simulink model "RonTrap_fig11"  (R2022b)
settings: Solver=ode15s  StartTime=-14  StopTime=39  MaxStep=0.025  RelTol=1e-7  AbsTol=1e-8
settings Model: Creator=Greatlovers  LastModifiedBy=Greatlovers

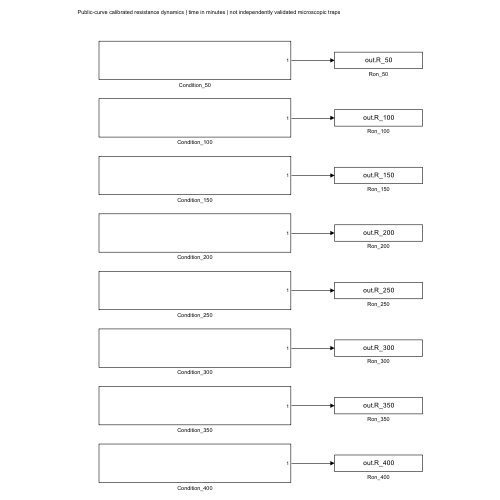
[thumbnail: Simulink's stored preview of the top-level diagram]
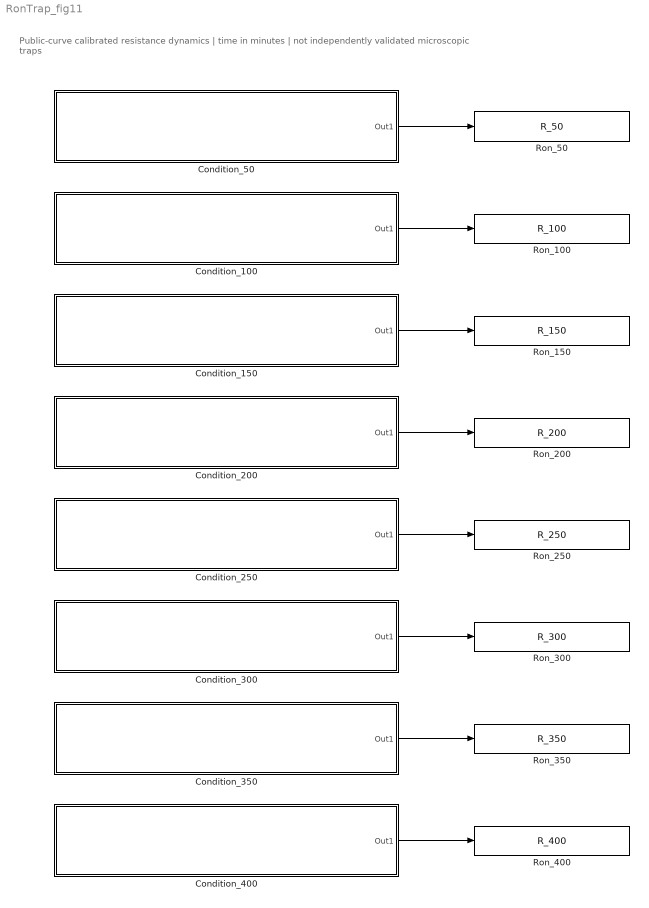
== system RonTrap_fig11 ==
  note: Public-curve calibrated resistance dynamics | time in minutes | not independently validated microscopic traps
  Condition_100 : Subsystem
  Condition_150 : Subsystem
  Condition_200 : Subsystem
  Condition_250 : Subsystem
  Condition_300 : Subsystem
  Condition_350 : Subsystem
  Condition_400 : Subsystem
  Condition_50 : Subsystem
  Ron_100 : ToWorkspace  VariableName=R_100  SaveFormat=Timeseries  SampleTime=-1
  Ron_150 : ToWorkspace  VariableName=R_150  SaveFormat=Timeseries  SampleTime=-1
  Ron_200 : ToWorkspace  VariableName=R_200  SaveFormat=Timeseries  SampleTime=-1
  Ron_250 : ToWorkspace  VariableName=R_250  SaveFormat=Timeseries  SampleTime=-1
  Ron_300 : ToWorkspace  VariableName=R_300  SaveFormat=Timeseries  SampleTime=-1
  Ron_350 : ToWorkspace  VariableName=R_350  SaveFormat=Timeseries  SampleTime=-1
  Ron_400 : ToWorkspace  VariableName=R_400  SaveFormat=Timeseries  SampleTime=-1
  Ron_50 : ToWorkspace  VariableName=R_50  SaveFormat=Timeseries  SampleTime=-1
  wires:
  Condition_50/1(Out1) -> Ron_50/1
  Condition_100/1(Out1) -> Ron_100/1
  Condition_150/1(Out1) -> Ron_150/1
  Condition_200/1(Out1) -> Ron_200/1
  Condition_250/1(Out1) -> Ron_250/1
  Condition_300/1(Out1) -> Ron_300/1
  Condition_350/1(Out1) -> Ron_350/1
  Condition_400/1(Out1) -> Ron_400/1

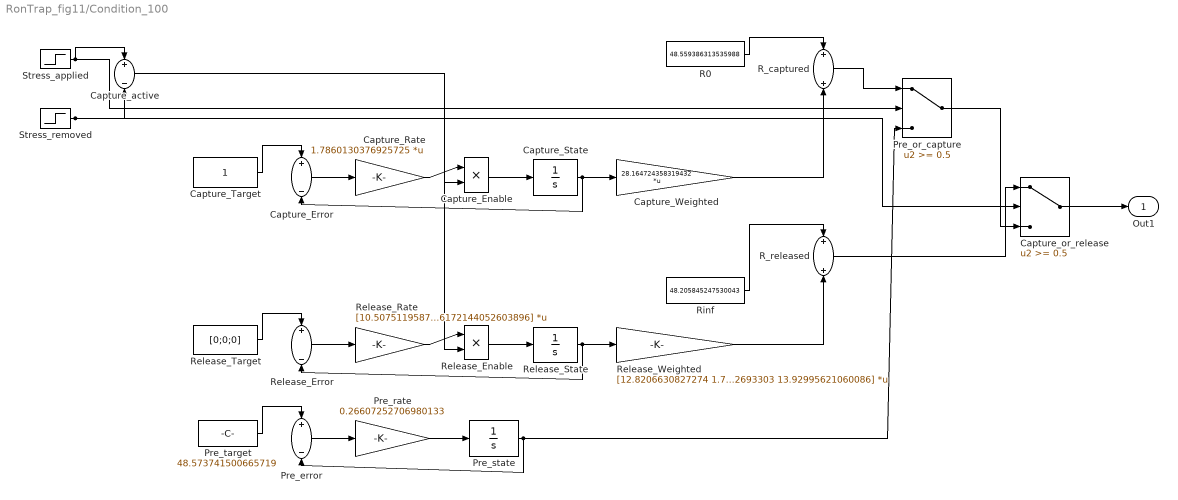
== system RonTrap_fig11/Condition_100 ==
  Capture_Enable : Product  Inputs=**
  Capture_Error : Sum  Inputs=+-
  Capture_Rate : Gain  Gain=1.7860130376925725  Multiplication=Matrix(K*u)
  Capture_State : Integrator
  Capture_Target : Constant
  Capture_Weighted : Gain  Gain=28.164724358319432  Multiplication=Matrix(K*u)
  Capture_active : Sum  Inputs=+-
  Capture_or_release : Switch  Threshold=0.5  SaturateOnIntegerOverflow=off  InputSameDT=off
  Pre_error : Sum  Inputs=+-
  Pre_or_capture : Switch  Threshold=0.5  SaturateOnIntegerOverflow=off  InputSameDT=off
  Pre_rate : Gain  Gain=0.26607252706980133
  Pre_state : Integrator  InitialCondition=47.988871358880552
  Pre_target : Constant  Value=48.573741500665719
  R0 : Constant  Value=48.559386313535988
  R_captured : Sum
  R_released : Sum
  Release_Enable : Product  Inputs=**
  Release_Error : Sum  Inputs=+-
  Release_Rate : Gain  Gain=[10.507511958742391 0 0;0 1.8533079959155121 0;0 0 0.26172144052603896]  Multiplication=Matrix(K*u)
  Release_State : Integrator  InitialCondition=[1;1;1]
  Release_Target : Constant  Value=[0;0;0]
  Release_Weighted : Gain  Gain=[12.8206630827274 1.7676461302693303 13.92995621060086]  Multiplication=Matrix(K*u)
  Rinf : Constant  Value=48.205845247530043
  Stress_applied : Step  Time=-0.066661845105779466  SampleTime=0
  Stress_removed : Step  Time=13.58333875417734  SampleTime=0
  Out1 : Outport
  wires:
  Stress_applied/1 -> Capture_active/1, Pre_or_capture/2
  Stress_removed/1 -> Capture_active/2, Release_Enable/2, Capture_or_release/2
  Capture_Target/1 -> Capture_Error/1
  Capture_State/1 -> Capture_Error/2, Capture_Weighted/1
  Capture_Error/1 -> Capture_Rate/1
  Capture_Rate/1 -> Capture_Enable/1
  Capture_Enable/1 -> Capture_State/1
  Release_Target/1 -> Release_Error/1
  Release_State/1 -> Release_Error/2, Release_Weighted/1
  Release_Error/1 -> Release_Rate/1
  Release_Rate/1 -> Release_Enable/1
  Release_Enable/1 -> Release_State/1
  Capture_active/1 -> Capture_Enable/2
  R0/1 -> R_captured/1
  Capture_Weighted/1 -> R_captured/2
  Rinf/1 -> R_released/1
  Release_Weighted/1 -> R_released/2
  Pre_target/1 -> Pre_error/1
  Pre_state/1 -> Pre_error/2, Pre_or_capture/3
  Pre_error/1 -> Pre_rate/1
  Pre_rate/1 -> Pre_state/1
  R_captured/1 -> Pre_or_capture/1
  R_released/1 -> Capture_or_release/1
  Pre_or_capture/1 -> Capture_or_release/3
  Capture_or_release/1 -> Out1/1

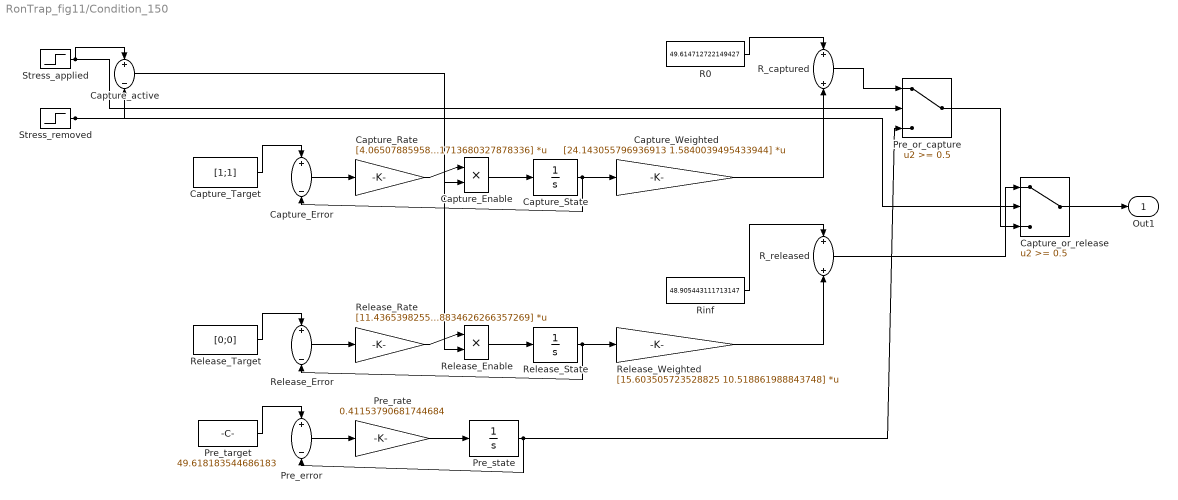
== system RonTrap_fig11/Condition_150 ==
  Capture_Enable : Product  Inputs=**
  Capture_Error : Sum  Inputs=+-
  Capture_Rate : Gain  Gain=[4.0650788595808649 0;0 0.11713680327878336]  Multiplication=Matrix(K*u)
  Capture_State : Integrator  InitialCondition=[0;0]
  Capture_Target : Constant  Value=[1;1]
  Capture_Weighted : Gain  Gain=[24.143055796936913 1.5840039495433944]  Multiplication=Matrix(K*u)
  Capture_active : Sum  Inputs=+-
  Capture_or_release : Switch  Threshold=0.5  SaturateOnIntegerOverflow=off  InputSameDT=off
  Pre_error : Sum  Inputs=+-
  Pre_or_capture : Switch  Threshold=0.5  SaturateOnIntegerOverflow=off  InputSameDT=off
  Pre_rate : Gain  Gain=0.41153790681744684
  Pre_state : Integrator  InitialCondition=48.544888767437868
  Pre_target : Constant  Value=49.618183544686183
  R0 : Constant  Value=49.614712722149427
  R_captured : Sum
  R_released : Sum
  Release_Enable : Product  Inputs=**
  Release_Error : Sum  Inputs=+-
  Release_Rate : Gain  Gain=[11.436539825510469 0;0 0.38834626266357269]  Multiplication=Matrix(K*u)
  Release_State : Integrator  InitialCondition=[1;1]
  Release_Target : Constant  Value=[0;0]
  Release_Weighted : Gain  Gain=[15.603505723528825 10.518861988843748]  Multiplication=Matrix(K*u)
  Rinf : Constant  Value=48.905443111713147
  Stress_applied : Step  Time=-0.066661845105779466  SampleTime=0
  Stress_removed : Step  Time=13.75000544608282  SampleTime=0
  Out1 : Outport
  wires:
  Stress_applied/1 -> Capture_active/1, Pre_or_capture/2
  Stress_removed/1 -> Capture_active/2, Release_Enable/2, Capture_or_release/2
  Capture_Target/1 -> Capture_Error/1
  Capture_State/1 -> Capture_Error/2, Capture_Weighted/1
  Capture_Error/1 -> Capture_Rate/1
  Capture_Rate/1 -> Capture_Enable/1
  Capture_Enable/1 -> Capture_State/1
  Release_Target/1 -> Release_Error/1
  Release_State/1 -> Release_Error/2, Release_Weighted/1
  Release_Error/1 -> Release_Rate/1
  Release_Rate/1 -> Release_Enable/1
  Release_Enable/1 -> Release_State/1
  Capture_active/1 -> Capture_Enable/2
  R0/1 -> R_captured/1
  Capture_Weighted/1 -> R_captured/2
  Rinf/1 -> R_released/1
  Release_Weighted/1 -> R_released/2
  Pre_target/1 -> Pre_error/1
  Pre_state/1 -> Pre_error/2, Pre_or_capture/3
  Pre_error/1 -> Pre_rate/1
  Pre_rate/1 -> Pre_state/1
  R_captured/1 -> Pre_or_capture/1
  R_released/1 -> Capture_or_release/1
  Pre_or_capture/1 -> Capture_or_release/3
  Capture_or_release/1 -> Out1/1

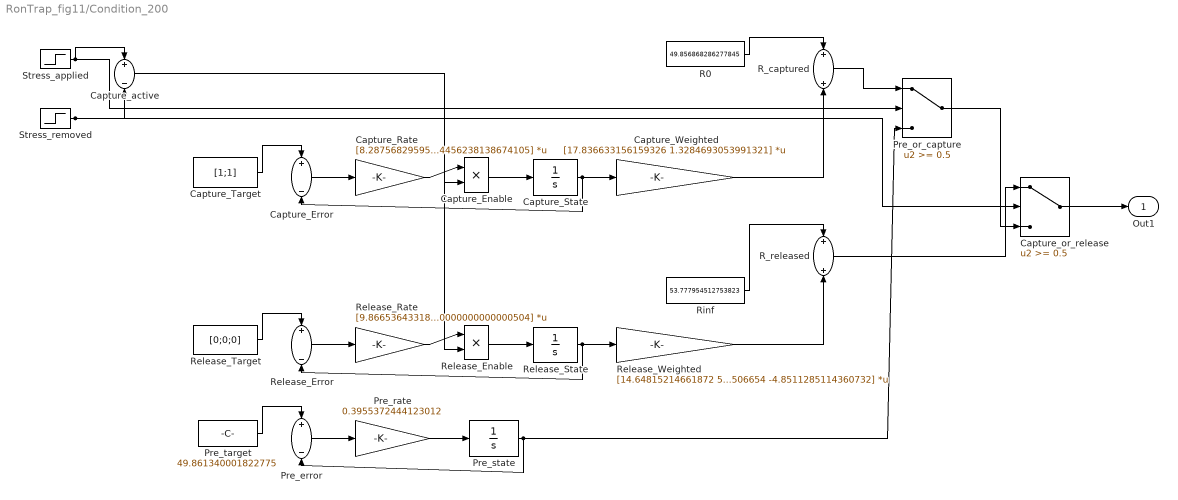
== system RonTrap_fig11/Condition_200 ==
  Capture_Enable : Product  Inputs=**
  Capture_Error : Sum  Inputs=+-
  Capture_Rate : Gain  Gain=[8.2875682959517381 0;0 0.24456238138674105]  Multiplication=Matrix(K*u)
  Capture_State : Integrator  InitialCondition=[0;0]
  Capture_Target : Constant  Value=[1;1]
  Capture_Weighted : Gain  Gain=[17.836633156159326 1.3284693053991321]  Multiplication=Matrix(K*u)
  Capture_active : Sum  Inputs=+-
  Capture_or_release : Switch  Threshold=0.5  SaturateOnIntegerOverflow=off  InputSameDT=off
  Pre_error : Sum  Inputs=+-
  Pre_or_capture : Switch  Threshold=0.5  SaturateOnIntegerOverflow=off  InputSameDT=off
  Pre_rate : Gain  Gain=0.3955372444123012
  Pre_state : Integrator  InitialCondition=48.754874141724315
  Pre_target : Constant  Value=49.861340001822775
  R0 : Constant  Value=49.856868286277845
  R_captured : Sum
  R_released : Sum
  Release_Enable : Product  Inputs=**
  Release_Error : Sum  Inputs=+-
  Release_Rate : Gain  Gain=[9.8665364331893439 0 0;0 0.56043585020711861 0;0 0 0.0050000000000000504]  Multiplication=Matrix(K*u)
  Release_State : Integrator  InitialCondition=[1;1;1]
  Release_Target : Constant  Value=[0;0;0]
  Release_Weighted : Gain  Gain=[14.64815214661872 5.4009738116506654 -4.8511285114360732]  Multiplication=Matrix(K*u)
  Rinf : Constant  Value=53.777954512753823
  Stress_applied : Step  Time=-0.066661845105779466  SampleTime=0
  Stress_removed : Step  Time=13.683338820821518  SampleTime=0
  Out1 : Outport
  wires:
  Stress_applied/1 -> Capture_active/1, Pre_or_capture/2
  Stress_removed/1 -> Capture_active/2, Release_Enable/2, Capture_or_release/2
  Capture_Target/1 -> Capture_Error/1
  Capture_State/1 -> Capture_Error/2, Capture_Weighted/1
  Capture_Error/1 -> Capture_Rate/1
  Capture_Rate/1 -> Capture_Enable/1
  Capture_Enable/1 -> Capture_State/1
  Release_Target/1 -> Release_Error/1
  Release_State/1 -> Release_Error/2, Release_Weighted/1
  Release_Error/1 -> Release_Rate/1
  Release_Rate/1 -> Release_Enable/1
  Release_Enable/1 -> Release_State/1
  Capture_active/1 -> Capture_Enable/2
  R0/1 -> R_captured/1
  Capture_Weighted/1 -> R_captured/2
  Rinf/1 -> R_released/1
  Release_Weighted/1 -> R_released/2
  Pre_target/1 -> Pre_error/1
  Pre_state/1 -> Pre_error/2, Pre_or_capture/3
  Pre_error/1 -> Pre_rate/1
  Pre_rate/1 -> Pre_state/1
  R_captured/1 -> Pre_or_capture/1
  R_released/1 -> Capture_or_release/1
  Pre_or_capture/1 -> Capture_or_release/3
  Capture_or_release/1 -> Out1/1

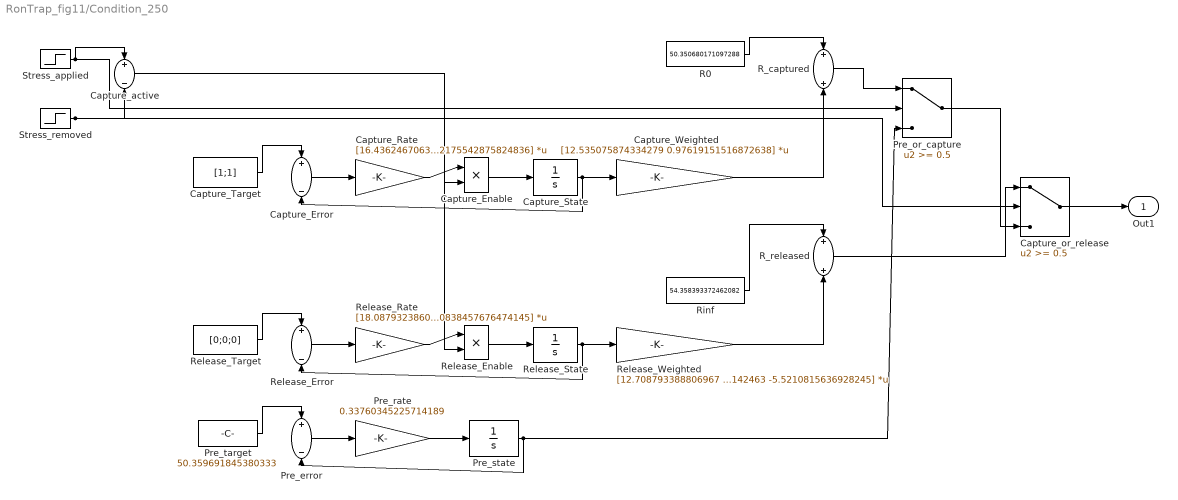
== system RonTrap_fig11/Condition_250 ==
  Capture_Enable : Product  Inputs=**
  Capture_Error : Sum  Inputs=+-
  Capture_Rate : Gain  Gain=[16.436246706364585 0;0 0.22175542875824836]  Multiplication=Matrix(K*u)
  Capture_State : Integrator  InitialCondition=[0;0]
  Capture_Target : Constant  Value=[1;1]
  Capture_Weighted : Gain  Gain=[12.535075874334279 0.97619151516872638]  Multiplication=Matrix(K*u)
  Capture_active : Sum  Inputs=+-
  Capture_or_release : Switch  Threshold=0.5  SaturateOnIntegerOverflow=off  InputSameDT=off
  Pre_error : Sum  Inputs=+-
  Pre_or_capture : Switch  Threshold=0.5  SaturateOnIntegerOverflow=off  InputSameDT=off
  Pre_rate : Gain  Gain=0.33760345225714189
  Pre_state : Integrator  InitialCondition=49.370550496010729
  Pre_target : Constant  Value=50.359691845380333
  R0 : Constant  Value=50.350680171097288
  R_captured : Sum
  R_released : Sum
  Release_Enable : Product  Inputs=**
  Release_Error : Sum  Inputs=+-
  Release_Rate : Gain  Gain=[18.087932386014803 0 0;0 1.0493415826811785 0;0 0 0.010838457676474145]  Multiplication=Matrix(K*u)
  Release_State : Integrator  InitialCondition=[1;1;1]
  Release_Target : Constant  Value=[0;0;0]
  Release_Weighted : Gain  Gain=[12.708793388806967 2.2685335284142463 -5.5210815636928245]  Multiplication=Matrix(K*u)
  Rinf : Constant  Value=54.358393372462082
  Stress_applied : Step  Time=-0.08332843704497743  SampleTime=0
  Stress_removed : Step  Time=13.566672162238142  SampleTime=0
  Out1 : Outport
  wires:
  Stress_applied/1 -> Capture_active/1, Pre_or_capture/2
  Stress_removed/1 -> Capture_active/2, Release_Enable/2, Capture_or_release/2
  Capture_Target/1 -> Capture_Error/1
  Capture_State/1 -> Capture_Error/2, Capture_Weighted/1
  Capture_Error/1 -> Capture_Rate/1
  Capture_Rate/1 -> Capture_Enable/1
  Capture_Enable/1 -> Capture_State/1
  Release_Target/1 -> Release_Error/1
  Release_State/1 -> Release_Error/2, Release_Weighted/1
  Release_Error/1 -> Release_Rate/1
  Release_Rate/1 -> Release_Enable/1
  Release_Enable/1 -> Release_State/1
  Capture_active/1 -> Capture_Enable/2
  R0/1 -> R_captured/1
  Capture_Weighted/1 -> R_captured/2
  Rinf/1 -> R_released/1
  Release_Weighted/1 -> R_released/2
  Pre_target/1 -> Pre_error/1
  Pre_state/1 -> Pre_error/2, Pre_or_capture/3
  Pre_error/1 -> Pre_rate/1
  Pre_rate/1 -> Pre_state/1
  R_captured/1 -> Pre_or_capture/1
  R_released/1 -> Capture_or_release/1
  Pre_or_capture/1 -> Capture_or_release/3
  Capture_or_release/1 -> Out1/1

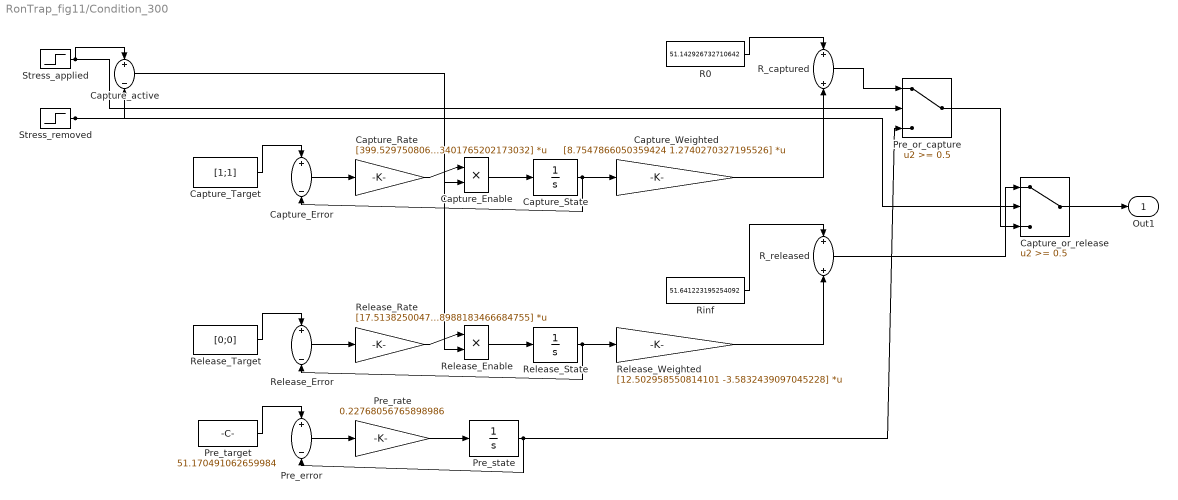
== system RonTrap_fig11/Condition_300 ==
  Capture_Enable : Product  Inputs=**
  Capture_Error : Sum  Inputs=+-
  Capture_Rate : Gain  Gain=[399.52975080658223 0;0 0.053401765202173032]  Multiplication=Matrix(K*u)
  Capture_State : Integrator  InitialCondition=[0;0]
  Capture_Target : Constant  Value=[1;1]
  Capture_Weighted : Gain  Gain=[8.7547866050359424 1.2740270327195526]  Multiplication=Matrix(K*u)
  Capture_active : Sum  Inputs=+-
  Capture_or_release : Switch  Threshold=0.5  SaturateOnIntegerOverflow=off  InputSameDT=off
  Pre_error : Sum  Inputs=+-
  Pre_or_capture : Switch  Threshold=0.5  SaturateOnIntegerOverflow=off  InputSameDT=off
  Pre_rate : Gain  Gain=0.22768056765898986
  Pre_state : Integrator  InitialCondition=50.512709513389304
  Pre_target : Constant  Value=51.170491062659984
  R0 : Constant  Value=51.142926732710642
  R_captured : Sum
  R_released : Sum
  Release_Enable : Product  Inputs=**
  Release_Error : Sum  Inputs=+-
  Release_Rate : Gain  Gain=[17.513825004745215 0;0 0.068988183466684755]  Multiplication=Matrix(K*u)
  Release_State : Integrator  InitialCondition=[1;1]
  Release_Target : Constant  Value=[0;0]
  Release_Weighted : Gain  Gain=[12.502958550814101 -3.5832439097045228]  Multiplication=Matrix(K*u)
  Rinf : Constant  Value=51.641223195254092
  Stress_applied : Step  Time=-0.066661845105779466  SampleTime=0
  Stress_removed : Step  Time=13.700005412760731  SampleTime=0
  Out1 : Outport
  wires:
  Stress_applied/1 -> Capture_active/1, Pre_or_capture/2
  Stress_removed/1 -> Capture_active/2, Release_Enable/2, Capture_or_release/2
  Capture_Target/1 -> Capture_Error/1
  Capture_State/1 -> Capture_Error/2, Capture_Weighted/1
  Capture_Error/1 -> Capture_Rate/1
  Capture_Rate/1 -> Capture_Enable/1
  Capture_Enable/1 -> Capture_State/1
  Release_Target/1 -> Release_Error/1
  Release_State/1 -> Release_Error/2, Release_Weighted/1
  Release_Error/1 -> Release_Rate/1
  Release_Rate/1 -> Release_Enable/1
  Release_Enable/1 -> Release_State/1
  Capture_active/1 -> Capture_Enable/2
  R0/1 -> R_captured/1
  Capture_Weighted/1 -> R_captured/2
  Rinf/1 -> R_released/1
  Release_Weighted/1 -> R_released/2
  Pre_target/1 -> Pre_error/1
  Pre_state/1 -> Pre_error/2, Pre_or_capture/3
  Pre_error/1 -> Pre_rate/1
  Pre_rate/1 -> Pre_state/1
  R_captured/1 -> Pre_or_capture/1
  R_released/1 -> Capture_or_release/1
  Pre_or_capture/1 -> Capture_or_release/3
  Capture_or_release/1 -> Out1/1

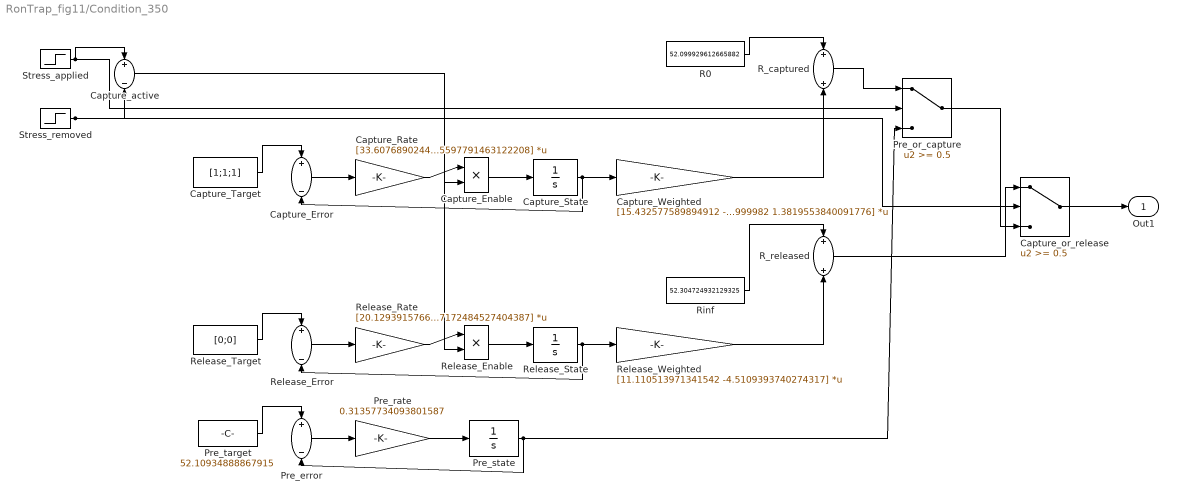
== system RonTrap_fig11/Condition_350 ==
  Capture_Enable : Product  Inputs=**
  Capture_Error : Sum  Inputs=+-
  Capture_Rate : Gain  Gain=[33.607689024482951 0 0;0 9.1903876408165228 0;0 0 0.35597791463122208]  Multiplication=Matrix(K*u)
  Capture_State : Integrator  InitialCondition=[0;0;0]
  Capture_Target : Constant  Value=[1;1;1]
  Capture_Weighted : Gain  Gain=[15.432577589894912 -9.9999999999999982 1.3819553840091776]  Multiplication=Matrix(K*u)
  Capture_active : Sum  Inputs=+-
  Capture_or_release : Switch  Threshold=0.5  SaturateOnIntegerOverflow=off  InputSameDT=off
  Pre_error : Sum  Inputs=+-
  Pre_or_capture : Switch  Threshold=0.5  SaturateOnIntegerOverflow=off  InputSameDT=off
  Pre_rate : Gain  Gain=0.31357734093801587
  Pre_state : Integrator  InitialCondition=51.369303816485981
  Pre_target : Constant  Value=52.10934888867915
  R0 : Constant  Value=52.099929612665882
  R_captured : Sum
  R_released : Sum
  Release_Enable : Product  Inputs=**
  Release_Error : Sum  Inputs=+-
  Release_Rate : Gain  Gain=[20.129391576645695 0;0 0.097172484527404387]  Multiplication=Matrix(K*u)
  Release_State : Integrator  InitialCondition=[1;1]
  Release_Target : Constant  Value=[0;0]
  Release_Weighted : Gain  Gain=[11.110513971341542 -4.5109393740274317]  Multiplication=Matrix(K*u)
  Rinf : Constant  Value=52.304724932129325
  Stress_applied : Step  Time=-0.08332843704497743  SampleTime=0
  Stress_removed : Step  Time=13.716672133452184  SampleTime=0
  Out1 : Outport
  wires:
  Stress_applied/1 -> Capture_active/1, Pre_or_capture/2
  Stress_removed/1 -> Capture_active/2, Release_Enable/2, Capture_or_release/2
  Capture_Target/1 -> Capture_Error/1
  Capture_State/1 -> Capture_Error/2, Capture_Weighted/1
  Capture_Error/1 -> Capture_Rate/1
  Capture_Rate/1 -> Capture_Enable/1
  Capture_Enable/1 -> Capture_State/1
  Release_Target/1 -> Release_Error/1
  Release_State/1 -> Release_Error/2, Release_Weighted/1
  Release_Error/1 -> Release_Rate/1
  Release_Rate/1 -> Release_Enable/1
  Release_Enable/1 -> Release_State/1
  Capture_active/1 -> Capture_Enable/2
  R0/1 -> R_captured/1
  Capture_Weighted/1 -> R_captured/2
  Rinf/1 -> R_released/1
  Release_Weighted/1 -> R_released/2
  Pre_target/1 -> Pre_error/1
  Pre_state/1 -> Pre_error/2, Pre_or_capture/3
  Pre_error/1 -> Pre_rate/1
  Pre_rate/1 -> Pre_state/1
  R_captured/1 -> Pre_or_capture/1
  R_released/1 -> Capture_or_release/1
  Pre_or_capture/1 -> Capture_or_release/3
  Capture_or_release/1 -> Out1/1

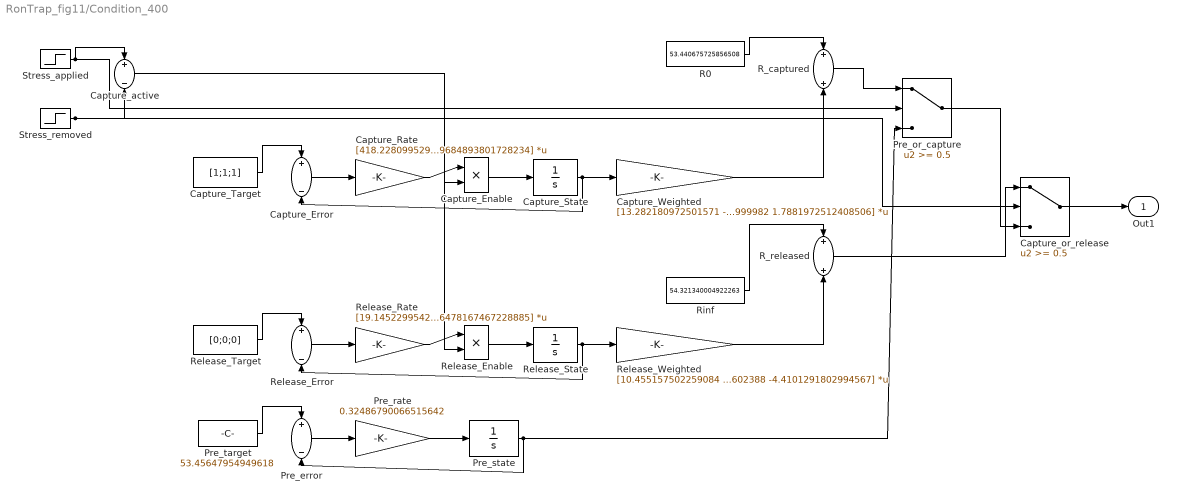
== system RonTrap_fig11/Condition_400 ==
  Capture_Enable : Product  Inputs=**
  Capture_Error : Sum  Inputs=+-
  Capture_Rate : Gain  Gain=[418.22809952967282 0 0;0 11.853248568471619 0;0 0 0.59684893801728234]  Multiplication=Matrix(K*u)
  Capture_State : Integrator  InitialCondition=[0;0;0]
  Capture_Target : Constant  Value=[1;1;1]
  Capture_Weighted : Gain  Gain=[13.282180972501571 -9.9999999999999982 1.7881972512408506]  Multiplication=Matrix(K*u)
  Capture_active : Sum  Inputs=+-
  Capture_or_release : Switch  Threshold=0.5  SaturateOnIntegerOverflow=off  InputSameDT=off
  Pre_error : Sum  Inputs=+-
  Pre_or_capture : Switch  Threshold=0.5  SaturateOnIntegerOverflow=off  InputSameDT=off
  Pre_rate : Gain  Gain=0.32486790066515642
  Pre_state : Integrator  InitialCondition=51.995669734255074
  Pre_target : Constant  Value=53.45647954949618
  R0 : Constant  Value=53.440675725856508
  R_captured : Sum
  R_released : Sum
  Release_Enable : Product  Inputs=**
  Release_Error : Sum  Inputs=+-
  Release_Rate : Gain  Gain=[19.145229954221044 0 0;0 0.4653580347126749 0;0 0 0.066478167467228885]  Multiplication=Matrix(K*u)
  Release_State : Integrator  InitialCondition=[1;1;1]
  Release_Target : Constant  Value=[0;0;0]
  Release_Weighted : Gain  Gain=[10.455157502259084 -1.8558071227602388 -4.4101291802994567]  Multiplication=Matrix(K*u)
  Rinf : Constant  Value=54.321340004922263
  Stress_applied : Step  Time=-0.066661845105779466  SampleTime=0
  Stress_removed : Step  Time=13.66667210013008  SampleTime=0
  Out1 : Outport
  wires:
  Stress_applied/1 -> Capture_active/1, Pre_or_capture/2
  Stress_removed/1 -> Capture_active/2, Release_Enable/2, Capture_or_release/2
  Capture_Target/1 -> Capture_Error/1
  Capture_State/1 -> Capture_Error/2, Capture_Weighted/1
  Capture_Error/1 -> Capture_Rate/1
  Capture_Rate/1 -> Capture_Enable/1
  Capture_Enable/1 -> Capture_State/1
  Release_Target/1 -> Release_Error/1
  Release_State/1 -> Release_Error/2, Release_Weighted/1
  Release_Error/1 -> Release_Rate/1
  Release_Rate/1 -> Release_Enable/1
  Release_Enable/1 -> Release_State/1
  Capture_active/1 -> Capture_Enable/2
  R0/1 -> R_captured/1
  Capture_Weighted/1 -> R_captured/2
  Rinf/1 -> R_released/1
  Release_Weighted/1 -> R_released/2
  Pre_target/1 -> Pre_error/1
  Pre_state/1 -> Pre_error/2, Pre_or_capture/3
  Pre_error/1 -> Pre_rate/1
  Pre_rate/1 -> Pre_state/1
  R_captured/1 -> Pre_or_capture/1
  R_released/1 -> Capture_or_release/1
  Pre_or_capture/1 -> Capture_or_release/3
  Capture_or_release/1 -> Out1/1

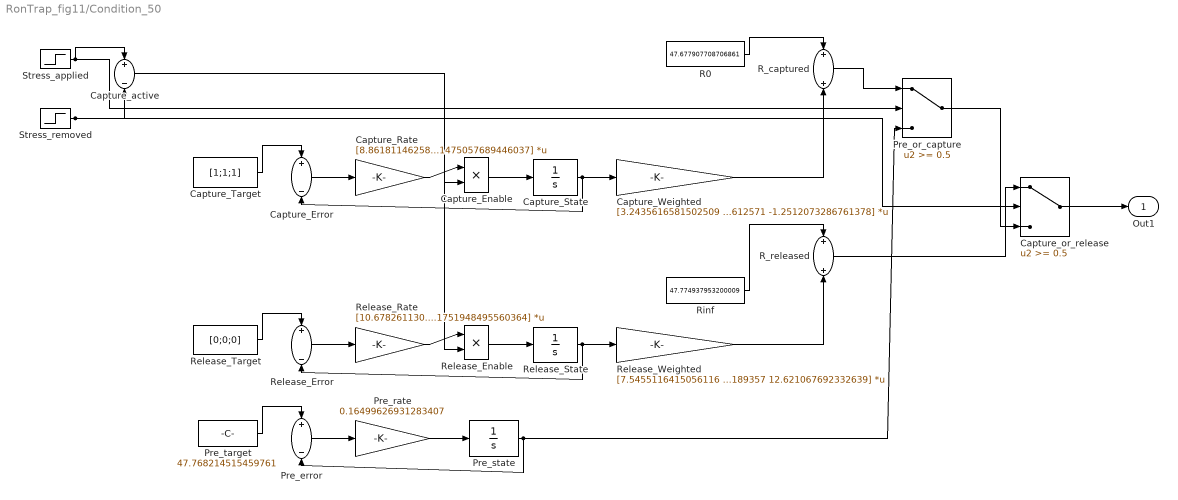
== system RonTrap_fig11/Condition_50 ==
  Capture_Enable : Product  Inputs=**
  Capture_Error : Sum  Inputs=+-
  Capture_Rate : Gain  Gain=[8.8618114625810875 0 0;0 0.66393851283050509 0;0 0 0.21475057689446037]  Multiplication=Matrix(K*u)
  Capture_State : Integrator  InitialCondition=[0;0;0]
  Capture_Target : Constant  Value=[1;1;1]
  Capture_Weighted : Gain  Gain=[3.2435616581502509 21.254439640612571 -1.2512073286761378]  Multiplication=Matrix(K*u)
  Capture_active : Sum  Inputs=+-
  Capture_or_release : Switch  Threshold=0.5  SaturateOnIntegerOverflow=off  InputSameDT=off
  Pre_error : Sum  Inputs=+-
  Pre_or_capture : Switch  Threshold=0.5  SaturateOnIntegerOverflow=off  InputSameDT=off
  Pre_rate : Gain  Gain=0.16499626931283407
  Pre_state : Integrator  InitialCondition=46.868424291616599
  Pre_target : Constant  Value=47.768214515459761
  R0 : Constant  Value=47.677907708706861
  R_captured : Sum
  R_released : Sum
  Release_Enable : Product  Inputs=**
  Release_Error : Sum  Inputs=+-
  Release_Rate : Gain  Gain=[10.678261130657335 0 0;0 1.0139554613764425 0;0 0 0.1751948495560364]  Multiplication=Matrix(K*u)
  Release_State : Integrator  InitialCondition=[1;1;1]
  Release_Target : Constant  Value=[0;0;0]
  Release_Weighted : Gain  Gain=[7.5455116415056116 3.0466001228189357 12.621067692332639]  Multiplication=Matrix(K*u)
  Rinf : Constant  Value=47.774937953200009
  Stress_applied : Step  Time=-0.066661845105779466  SampleTime=0
  Stress_removed : Step  Time=13.650005379438626  SampleTime=0
  Out1 : Outport
  wires:
  Stress_applied/1 -> Capture_active/1, Pre_or_capture/2
  Stress_removed/1 -> Capture_active/2, Release_Enable/2, Capture_or_release/2
  Capture_Target/1 -> Capture_Error/1
  Capture_State/1 -> Capture_Error/2, Capture_Weighted/1
  Capture_Error/1 -> Capture_Rate/1
  Capture_Rate/1 -> Capture_Enable/1
  Capture_Enable/1 -> Capture_State/1
  Release_Target/1 -> Release_Error/1
  Release_State/1 -> Release_Error/2, Release_Weighted/1
  Release_Error/1 -> Release_Rate/1
  Release_Rate/1 -> Release_Enable/1
  Release_Enable/1 -> Release_State/1
  Capture_active/1 -> Capture_Enable/2
  R0/1 -> R_captured/1
  Capture_Weighted/1 -> R_captured/2
  Rinf/1 -> R_released/1
  Release_Weighted/1 -> R_released/2
  Pre_target/1 -> Pre_error/1
  Pre_state/1 -> Pre_error/2, Pre_or_capture/3
  Pre_error/1 -> Pre_rate/1
  Pre_rate/1 -> Pre_state/1
  R_captured/1 -> Pre_or_capture/1
  R_released/1 -> Capture_or_release/1
  Pre_or_capture/1 -> Capture_or_release/3
  Capture_or_release/1 -> Out1/1
